simulink model "MOBATSim"  (R2020b)
settings: Solver=FixedStepAuto  StartTime=0.0  StopTime=Sim_t  FixedStep=0.01  MinStep=0.01  RelTol=1e-2
values from neighbouring files (symbols this model uses):
  Vehicles = evalin('base','Vehicles')    [I2V.m]    (also in VehicleSensors.m)
undefined symbols (not defined in the file or in its folder): Sim_Ts
libraries: simulink x50, robotalgslib x10, drivingvehiclecontroller x10, mpcadaslib x10, pid_lib x10
(part 6 of 7)

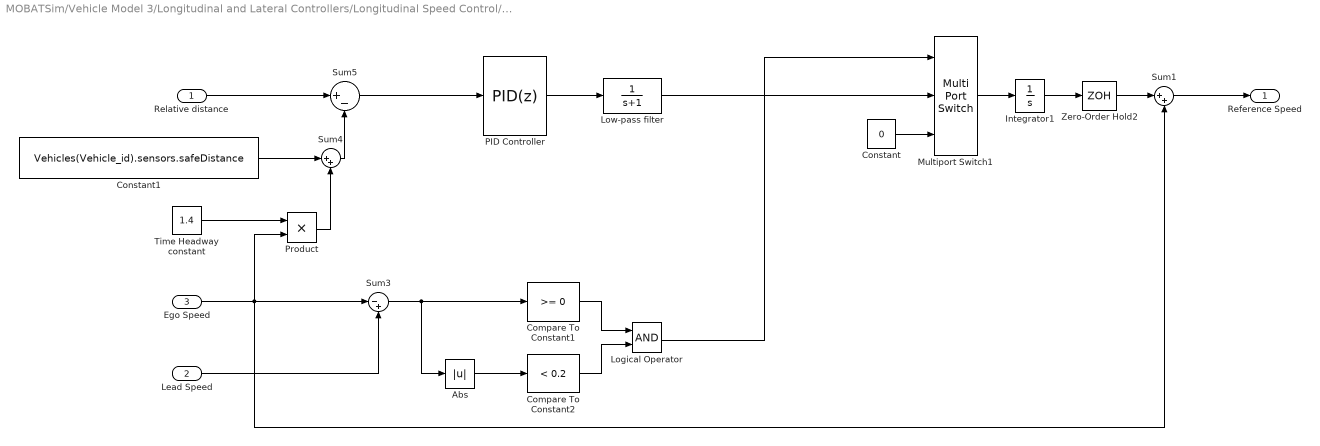
== system MOBATSim/Vehicle Model 3/Longitudinal and Lateral Controllers/Longitudinal Speed Control/Longitudinal Distance Control/PID-based ==
  Relative distance : Inport
  Lead Speed : Inport  Port=2
  Ego Speed : Inport  Port=3
  Abs : Abs
  Compare To Constant1 : simulink/Logic and Bit Operations/Compare To Constant  relop=>=  const=0  OutDataTypeStr=uint8
  Compare To Constant2 : simulink/Logic and Bit Operations/Compare To Constant  relop=<  const=0.2  OutDataTypeStr=uint8
  Constant : Constant  Value=0
  Constant1 : Constant  Value=Vehicles(Vehicle_id).sensors.safeDistance
  Integrator1 : Integrator  LimitOutput=on  UpperSaturationLimit=2  LowerSaturationLimit=-3
  Logical Operator : Logic  AllPortsSameDT=off  OutDataTypeStr=boolean
  Low-pass filter : TransferFcn  Denominator=[1 1]
  Multiport Switch1 : MultiPortSwitch  DataPortOrder=Zero-based contiguous  Inputs=2  zeroidx=on
  PID Controller : pid_lib/PID Controller  Controller=PID  Form=Parallel  TimeDomain=Discrete-time  UseExternalTs=off  SampleTime=0.1  IntegratorMethod=Trapezoidal  FilterMethod=Trapezoidal  ControllerParametersSource=internal  P=1.2  I=0.02  D=0.3  UseFilter=on  N=230  TunerSelectOption=Transfer Function Based (PID Tuner App)  InitialConditionSource=internal  InitialConditionForIntegrator=0  InitialConditionForFilter=0  DifferentiatorICPrevScaledInput=0  ExternalReset=none  TrackingMode=off  Kt=1  LimitOutput=on  SatLimitsSource=internal  UpperSaturationLimit=2  LowerSaturationLimit=-3  LinearizeAsGain=on  AntiWindupMode=back-calculation  Kb=1  POutMin=[]  POutMax=[]  IOutMin=[]  IOutMax=[]  DOutMin=[]  DOutMax=[]  NOutMin=[]  NOutMax=[]  SumOutMin=[]  SumOutMax=[]  SaturationOutMin=[]  SaturationOutMax=[]  PParamMin=[]  PParamMax=[]  IParamMin=[]  IParamMax=[]  DParamMin=[]  DParamMax=[]  NParamMin=[]  NParamMax=[]  KbParamMin=[]  KbParamMax=[]  KtParamMin=[]  KtParamMax=[]  KbOutMin=[]  KbOutMax=[]  KtOutMin=[]  KtOutMax=[]  IntegratorOutMin=[]  IntegratorOutMax=[]  FilterOutMin=[]  FilterOutMax=[]  SumI1OutMin=[]  SumI1OutMax=[]  SumI2OutMin=[]  SumI2OutMax=[]  SumI3OutMin=[]  SumI3OutMax=[]  SumI4OutMin=[]  SumI4OutMax=[]  SumDOutMin=[]  SumDOutMax=[]  DifferentiatorOutMin=[]  DifferentiatorOutMax=[]  FilterDiffOutCoefMin=[]  FilterDiffOutCoefMax=[]  ReciprocalOutMin=[]  ReciprocalOutMax=[]  SumDenOutMin=[]  SumDenOutMax=[]  SumNumOutMin=[]  SumNumOutMax=[]  DivideOutMin=[]  DivideOutMax=[]  UdiffTsProdOutMin=[]  UdiffTsProdOutMax=[]  NTsProdOutMin=[]  NTsProdOutMax=[]  UintegralTsProdOutMin=[]  UintegralTsProdOutMax=[]  UngainTsProdOutMin=[]  UngainTsProdOutMax=[]  IntegratorContinuousStateAttributes=''  IntegratorStateMustResolveToSignalObject=off  IntegratorRTWStateStorageClass=Auto  FilterContinuousStateAttributes=''  FilterStateMustResolveToSignalObject=off  FilterRTWStateStorageClass=Auto  ParallelPVariant=InternalParameters  IdealPVariant=Disabled  IVariant=InternalParameters  DVariant=InternalParameters  IntegratorVariant=Discrete  SatVariant=Enabled  AWVariant=BackCalculation  PCopyVariant=Disabled  TRVariant=Disabled  FdbkBlocksVariant=Feedback  IdealPFdbkVariant=Passthrough  SatFdbkVariant=Enabled  DerivativeFilterVariant=TrapezoidalFilter  NVariant=InternalParameters  NCopyVariant=InternalParameters  FilterICVariant=InternalICsFilter  IntegratorICVariant=InternalICs  ExternalResetVariant=Disabled  TRSumVariant=Passthrough  SumFdbkVariant=Enabled  SumVariant=Sum_PID  TsampFilterVariant=InternalTs  TsampNgainVariant=Passthrough  TsampIntegralVariant=Passthrough  ExternalSaturationOutDataTypeStr=Inherit: Same as second input
  Product : Product
  Sum1 : Sum  Inputs=|++
  Sum3 : Sum  Inputs=|-+
  Sum4 : Sum  Inputs=|++
  Sum5 : Sum  Inputs=|+-
  Time Headway constant : Constant  Value=1.4
  Zero-Order Hold2 : ZeroOrderHold  SampleTime=Sim_Ts
  Reference Speed : Outport  VectorParamsAs1DForOutWhenUnconnected=off
  wires:
  Low-pass filter/1 -> Multiport Switch1/2
  Lead Speed/1 -> Sum3/2
  PID Controller/1 -> Low-pass filter/1
  Time Headway constant/1 -> Product/1
  Constant1/1 -> Sum4/1
  Sum4/1 -> Sum5/2
  Abs/1 -> Compare To Constant2/1
  Logical Operator/1 -> Multiport Switch1/1
  Compare To Constant2/1 -> Logical Operator/2
  Sum5/1 -> PID Controller/1
  Constant/1 -> Multiport Switch1/3
  Product/1 -> Sum4/2
  Relative distance/1 -> Sum5/1
  Sum3/1 -> Abs/1, Compare To Constant1/1
  Compare To Constant1/1 -> Logical Operator/1
  Zero-Order Hold2/1 -> Sum1/1
  Ego Speed/1 -> Product/2, Sum1/2, Sum3/1
  Integrator1/1 -> Zero-Order Hold2/1
  Multiport Switch1/1 -> Integrator1/1
  Sum1/1 -> Reference Speed/1

== system MOBATSim/Vehicle Model 4/Longitudinal and Lateral Controllers/Lateral Motion Control/Pure Pursuit/Wheel Steering Angle Formulation ==
  note: $\delta(t)=tan^{-1} \left( \frac{2\ L\ sin(\alpha)}{l_{d}} \right)$
  alpha : Inport
  Atan : Trigonometry  Operator=atan
  Divide : Product  Inputs=*/
  Gain : Gain  Gain=2
  One over Look Ahead Distance : Constant  Value=6
  Product : Product
  Sine Wave : Sin  TimeSource=Use external signal  SampleTime=0
  Wheel Base : Constant  Value=3
  referenceYawAngle : Outport
  wires:
  Wheel Base/1 -> Gain/1
  Gain/1 -> Product/1
  alpha/1 -> Sine Wave/1
  Sine Wave/1 -> Product/2
  Product/1 -> Divide/1
  One over Look Ahead Distance/1 -> Divide/2
  Divide/1 -> Atan/1
  Atan/1 -> referenceYawAngle/1

== system MOBATSim/Vehicle Model 4/Longitudinal and Lateral Controllers/Longitudinal Speed Control/Longitudinal Distance Control/MPC-based ==
  note: Needs Model Predictive Control Toolbox™ to run
  Relative distance : Inport
  Lead Speed : Inport  Port=2
  Ego Speed : Inport  Port=3
  Adaptive Cruise Control System : mpcadaslib/Adaptive Cruise Control System  EgoModel=tf(1,[1,0])  InitialEgoVelocity=0  DefaultSpacing=Vehicles(Vehicle_id).sensors.safeDistance  MaxVelocity=Vehicles(Vehicle_id).dynamics.maxSpeed  MinAcceleration=-3  amin_ext=off  MaxAcceleration=2  amax_ext=off  Ts=0.4  PredictionHorizon=5  ControllerBehavior=0.620  suboptimal=off  maxiter=10  datatypeopt=double  optmode=off  trackmode=off
  Constant1 : Constant  Value=1.4
  Constant2 : Constant  Value=Vehicles(Vehicle_id).dynamics.maxSpeed
  Integrator1 : Integrator  LimitOutput=on  UpperSaturationLimit=2  LowerSaturationLimit=-3
  Sum : Sum  Inputs=|-+
  Sum4 : Sum  Inputs=|++
  Zero-Order Hold2 : ZeroOrderHold  SampleTime=Sim_Ts
  Reference Speed : Outport  VectorParamsAs1DForOutWhenUnconnected=off
  wires:
  Sum/1 -> Adaptive Cruise Control System/5
  Relative distance/1 -> Adaptive Cruise Control System/4
  Adaptive Cruise Control System/1 -> Integrator1/1
  Integrator1/1 -> Zero-Order Hold2/1
  Sum4/1 -> Reference Speed/1
  Constant1/1 -> Adaptive Cruise Control System/2
  Constant2/1 -> Adaptive Cruise Control System/1
  Lead Speed/1 -> Sum/2
  Ego Speed/1 -> Sum4/2, Adaptive Cruise Control System/3, Sum/1
  Zero-Order Hold2/1 -> Sum4/1

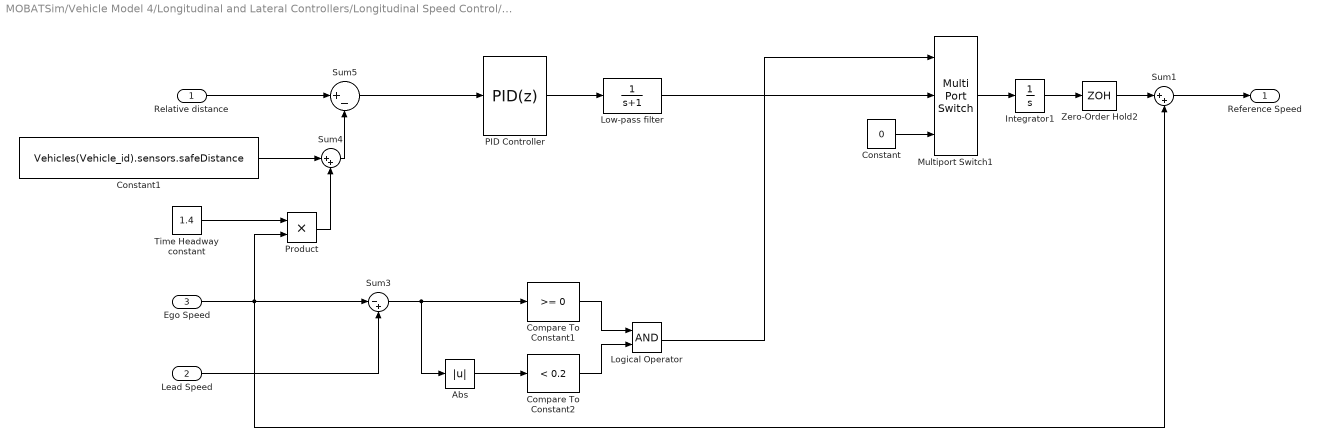
== system MOBATSim/Vehicle Model 4/Longitudinal and Lateral Controllers/Longitudinal Speed Control/Longitudinal Distance Control/PID-based ==
  Relative distance : Inport
  Lead Speed : Inport  Port=2
  Ego Speed : Inport  Port=3
  Abs : Abs
  Compare To Constant1 : simulink/Logic and Bit Operations/Compare To Constant  relop=>=  const=0  OutDataTypeStr=uint8
  Compare To Constant2 : simulink/Logic and Bit Operations/Compare To Constant  relop=<  const=0.2  OutDataTypeStr=uint8
  Constant : Constant  Value=0
  Constant1 : Constant  Value=Vehicles(Vehicle_id).sensors.safeDistance
  Integrator1 : Integrator  LimitOutput=on  UpperSaturationLimit=2  LowerSaturationLimit=-3
  Logical Operator : Logic  AllPortsSameDT=off  OutDataTypeStr=boolean
  Low-pass filter : TransferFcn  Denominator=[1 1]
  Multiport Switch1 : MultiPortSwitch  DataPortOrder=Zero-based contiguous  Inputs=2  zeroidx=on
  PID Controller : pid_lib/PID Controller  Controller=PID  Form=Parallel  TimeDomain=Discrete-time  UseExternalTs=off  SampleTime=0.1  IntegratorMethod=Trapezoidal  FilterMethod=Trapezoidal  ControllerParametersSource=internal  P=1.2  I=0.02  D=0.3  UseFilter=on  N=230  TunerSelectOption=Transfer Function Based (PID Tuner App)  InitialConditionSource=internal  InitialConditionForIntegrator=0  InitialConditionForFilter=0  DifferentiatorICPrevScaledInput=0  ExternalReset=none  TrackingMode=off  Kt=1  LimitOutput=on  SatLimitsSource=internal  UpperSaturationLimit=2  LowerSaturationLimit=-3  LinearizeAsGain=on  AntiWindupMode=back-calculation  Kb=1  POutMin=[]  POutMax=[]  IOutMin=[]  IOutMax=[]  DOutMin=[]  DOutMax=[]  NOutMin=[]  NOutMax=[]  SumOutMin=[]  SumOutMax=[]  SaturationOutMin=[]  SaturationOutMax=[]  PParamMin=[]  PParamMax=[]  IParamMin=[]  IParamMax=[]  DParamMin=[]  DParamMax=[]  NParamMin=[]  NParamMax=[]  KbParamMin=[]  KbParamMax=[]  KtParamMin=[]  KtParamMax=[]  KbOutMin=[]  KbOutMax=[]  KtOutMin=[]  KtOutMax=[]  IntegratorOutMin=[]  IntegratorOutMax=[]  FilterOutMin=[]  FilterOutMax=[]  SumI1OutMin=[]  SumI1OutMax=[]  SumI2OutMin=[]  SumI2OutMax=[]  SumI3OutMin=[]  SumI3OutMax=[]  SumI4OutMin=[]  SumI4OutMax=[]  SumDOutMin=[]  SumDOutMax=[]  DifferentiatorOutMin=[]  DifferentiatorOutMax=[]  FilterDiffOutCoefMin=[]  FilterDiffOutCoefMax=[]  ReciprocalOutMin=[]  ReciprocalOutMax=[]  SumDenOutMin=[]  SumDenOutMax=[]  SumNumOutMin=[]  SumNumOutMax=[]  DivideOutMin=[]  DivideOutMax=[]  UdiffTsProdOutMin=[]  UdiffTsProdOutMax=[]  NTsProdOutMin=[]  NTsProdOutMax=[]  UintegralTsProdOutMin=[]  UintegralTsProdOutMax=[]  UngainTsProdOutMin=[]  UngainTsProdOutMax=[]  IntegratorContinuousStateAttributes=''  IntegratorStateMustResolveToSignalObject=off  IntegratorRTWStateStorageClass=Auto  FilterContinuousStateAttributes=''  FilterStateMustResolveToSignalObject=off  FilterRTWStateStorageClass=Auto  ParallelPVariant=InternalParameters  IdealPVariant=Disabled  IVariant=InternalParameters  DVariant=InternalParameters  IntegratorVariant=Discrete  SatVariant=Enabled  AWVariant=BackCalculation  PCopyVariant=Disabled  TRVariant=Disabled  FdbkBlocksVariant=Feedback  IdealPFdbkVariant=Passthrough  SatFdbkVariant=Enabled  DerivativeFilterVariant=TrapezoidalFilter  NVariant=InternalParameters  NCopyVariant=InternalParameters  FilterICVariant=InternalICsFilter  IntegratorICVariant=InternalICs  ExternalResetVariant=Disabled  TRSumVariant=Passthrough  SumFdbkVariant=Enabled  SumVariant=Sum_PID  TsampFilterVariant=InternalTs  TsampNgainVariant=Passthrough  TsampIntegralVariant=Passthrough  ExternalSaturationOutDataTypeStr=Inherit: Same as second input
  Product : Product
  Sum1 : Sum  Inputs=|++
  Sum3 : Sum  Inputs=|-+
  Sum4 : Sum  Inputs=|++
  Sum5 : Sum  Inputs=|+-
  Time Headway constant : Constant  Value=1.4
  Zero-Order Hold2 : ZeroOrderHold  SampleTime=Sim_Ts
  Reference Speed : Outport  VectorParamsAs1DForOutWhenUnconnected=off
  wires:
  Low-pass filter/1 -> Multiport Switch1/2
  Lead Speed/1 -> Sum3/2
  PID Controller/1 -> Low-pass filter/1
  Time Headway constant/1 -> Product/1
  Constant1/1 -> Sum4/1
  Sum4/1 -> Sum5/2
  Abs/1 -> Compare To Constant2/1
  Logical Operator/1 -> Multiport Switch1/1
  Compare To Constant2/1 -> Logical Operator/2
  Sum5/1 -> PID Controller/1
  Constant/1 -> Multiport Switch1/3
  Product/1 -> Sum4/2
  Relative distance/1 -> Sum5/1
  Sum3/1 -> Abs/1, Compare To Constant1/1
  Compare To Constant1/1 -> Logical Operator/1
  Zero-Order Hold2/1 -> Sum1/1
  Ego Speed/1 -> Product/2, Sum1/2, Sum3/1
  Integrator1/1 -> Zero-Order Hold2/1
  Multiport Switch1/1 -> Integrator1/1
  Sum1/1 -> Reference Speed/1

== system MOBATSim/Vehicle Model 5/Longitudinal and Lateral Controllers/Lateral Motion Control/Pure Pursuit/Wheel Steering Angle Formulation ==
  note: $\delta(t)=tan^{-1} \left( \frac{2\ L\ sin(\alpha)}{l_{d}} \right)$
  alpha : Inport
  Atan : Trigonometry  Operator=atan
  Divide : Product  Inputs=*/
  Gain : Gain  Gain=2
  One over Look Ahead Distance : Constant  Value=6
  Product : Product
  Sine Wave : Sin  TimeSource=Use external signal  SampleTime=0
  Wheel Base : Constant  Value=3
  referenceYawAngle : Outport
  wires:
  Wheel Base/1 -> Gain/1
  Gain/1 -> Product/1
  alpha/1 -> Sine Wave/1
  Sine Wave/1 -> Product/2
  Product/1 -> Divide/1
  One over Look Ahead Distance/1 -> Divide/2
  Divide/1 -> Atan/1
  Atan/1 -> referenceYawAngle/1

== system MOBATSim/Vehicle Model 5/Longitudinal and Lateral Controllers/Longitudinal Speed Control/Longitudinal Distance Control/MPC-based ==
  note: Needs Model Predictive Control Toolbox™ to run
  Relative distance : Inport
  Lead Speed : Inport  Port=2
  Ego Speed : Inport  Port=3
  Adaptive Cruise Control System : mpcadaslib/Adaptive Cruise Control System  EgoModel=tf(1,[1,0])  InitialEgoVelocity=0  DefaultSpacing=Vehicles(Vehicle_id).sensors.safeDistance  MaxVelocity=Vehicles(Vehicle_id).dynamics.maxSpeed  MinAcceleration=-3  amin_ext=off  MaxAcceleration=2  amax_ext=off  Ts=0.4  PredictionHorizon=5  ControllerBehavior=0.620  suboptimal=off  maxiter=10  datatypeopt=double  optmode=off  trackmode=off
  Constant1 : Constant  Value=1.4
  Constant2 : Constant  Value=Vehicles(Vehicle_id).dynamics.maxSpeed
  Integrator1 : Integrator  LimitOutput=on  UpperSaturationLimit=2  LowerSaturationLimit=-3
  Sum : Sum  Inputs=|-+
  Sum4 : Sum  Inputs=|++
  Zero-Order Hold2 : ZeroOrderHold  SampleTime=Sim_Ts
  Reference Speed : Outport  VectorParamsAs1DForOutWhenUnconnected=off
  wires:
  Sum/1 -> Adaptive Cruise Control System/5
  Relative distance/1 -> Adaptive Cruise Control System/4
  Adaptive Cruise Control System/1 -> Integrator1/1
  Integrator1/1 -> Zero-Order Hold2/1
  Sum4/1 -> Reference Speed/1
  Constant1/1 -> Adaptive Cruise Control System/2
  Constant2/1 -> Adaptive Cruise Control System/1
  Lead Speed/1 -> Sum/2
  Ego Speed/1 -> Sum4/2, Adaptive Cruise Control System/3, Sum/1
  Zero-Order Hold2/1 -> Sum4/1

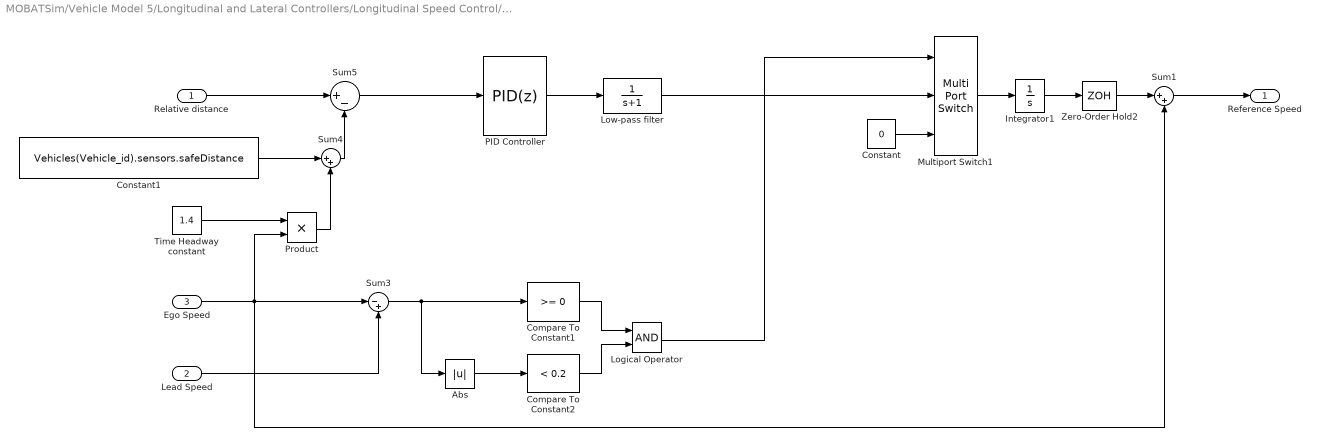
== system MOBATSim/Vehicle Model 5/Longitudinal and Lateral Controllers/Longitudinal Speed Control/Longitudinal Distance Control/PID-based ==
  Relative distance : Inport
  Lead Speed : Inport  Port=2
  Ego Speed : Inport  Port=3
  Abs : Abs
  Compare To Constant1 : simulink/Logic and Bit Operations/Compare To Constant  relop=>=  const=0  OutDataTypeStr=uint8
  Compare To Constant2 : simulink/Logic and Bit Operations/Compare To Constant  relop=<  const=0.2  OutDataTypeStr=uint8
  Constant : Constant  Value=0
  Constant1 : Constant  Value=Vehicles(Vehicle_id).sensors.safeDistance
  Integrator1 : Integrator  LimitOutput=on  UpperSaturationLimit=2  LowerSaturationLimit=-3
  Logical Operator : Logic  AllPortsSameDT=off  OutDataTypeStr=boolean
  Low-pass filter : TransferFcn  Denominator=[1 1]
  Multiport Switch1 : MultiPortSwitch  DataPortOrder=Zero-based contiguous  Inputs=2  zeroidx=on
  PID Controller : pid_lib/PID Controller  Controller=PID  Form=Parallel  TimeDomain=Discrete-time  UseExternalTs=off  SampleTime=0.1  IntegratorMethod=Trapezoidal  FilterMethod=Trapezoidal  ControllerParametersSource=internal  P=1.2  I=0.02  D=0.3  UseFilter=on  N=230  TunerSelectOption=Transfer Function Based (PID Tuner App)  InitialConditionSource=internal  InitialConditionForIntegrator=0  InitialConditionForFilter=0  DifferentiatorICPrevScaledInput=0  ExternalReset=none  TrackingMode=off  Kt=1  LimitOutput=on  SatLimitsSource=internal  UpperSaturationLimit=2  LowerSaturationLimit=-3  LinearizeAsGain=on  AntiWindupMode=back-calculation  Kb=1  POutMin=[]  POutMax=[]  IOutMin=[]  IOutMax=[]  DOutMin=[]  DOutMax=[]  NOutMin=[]  NOutMax=[]  SumOutMin=[]  SumOutMax=[]  SaturationOutMin=[]  SaturationOutMax=[]  PParamMin=[]  PParamMax=[]  IParamMin=[]  IParamMax=[]  DParamMin=[]  DParamMax=[]  NParamMin=[]  NParamMax=[]  KbParamMin=[]  KbParamMax=[]  KtParamMin=[]  KtParamMax=[]  KbOutMin=[]  KbOutMax=[]  KtOutMin=[]  KtOutMax=[]  IntegratorOutMin=[]  IntegratorOutMax=[]  FilterOutMin=[]  FilterOutMax=[]  SumI1OutMin=[]  SumI1OutMax=[]  SumI2OutMin=[]  SumI2OutMax=[]  SumI3OutMin=[]  SumI3OutMax=[]  SumI4OutMin=[]  SumI4OutMax=[]  SumDOutMin=[]  SumDOutMax=[]  DifferentiatorOutMin=[]  DifferentiatorOutMax=[]  FilterDiffOutCoefMin=[]  FilterDiffOutCoefMax=[]  ReciprocalOutMin=[]  ReciprocalOutMax=[]  SumDenOutMin=[]  SumDenOutMax=[]  SumNumOutMin=[]  SumNumOutMax=[]  DivideOutMin=[]  DivideOutMax=[]  UdiffTsProdOutMin=[]  UdiffTsProdOutMax=[]  NTsProdOutMin=[]  NTsProdOutMax=[]  UintegralTsProdOutMin=[]  UintegralTsProdOutMax=[]  UngainTsProdOutMin=[]  UngainTsProdOutMax=[]  IntegratorContinuousStateAttributes=''  IntegratorStateMustResolveToSignalObject=off  IntegratorRTWStateStorageClass=Auto  FilterContinuousStateAttributes=''  FilterStateMustResolveToSignalObject=off  FilterRTWStateStorageClass=Auto  ParallelPVariant=InternalParameters  IdealPVariant=Disabled  IVariant=InternalParameters  DVariant=InternalParameters  IntegratorVariant=Discrete  SatVariant=Enabled  AWVariant=BackCalculation  PCopyVariant=Disabled  TRVariant=Disabled  FdbkBlocksVariant=Feedback  IdealPFdbkVariant=Passthrough  SatFdbkVariant=Enabled  DerivativeFilterVariant=TrapezoidalFilter  NVariant=InternalParameters  NCopyVariant=InternalParameters  FilterICVariant=InternalICsFilter  IntegratorICVariant=InternalICs  ExternalResetVariant=Disabled  TRSumVariant=Passthrough  SumFdbkVariant=Enabled  SumVariant=Sum_PID  TsampFilterVariant=InternalTs  TsampNgainVariant=Passthrough  TsampIntegralVariant=Passthrough  ExternalSaturationOutDataTypeStr=Inherit: Same as second input
  Product : Product
  Sum1 : Sum  Inputs=|++
  Sum3 : Sum  Inputs=|-+
  Sum4 : Sum  Inputs=|++
  Sum5 : Sum  Inputs=|+-
  Time Headway constant : Constant  Value=1.4
  Zero-Order Hold2 : ZeroOrderHold  SampleTime=Sim_Ts
  Reference Speed : Outport  VectorParamsAs1DForOutWhenUnconnected=off
  wires:
  Low-pass filter/1 -> Multiport Switch1/2
  Lead Speed/1 -> Sum3/2
  PID Controller/1 -> Low-pass filter/1
  Time Headway constant/1 -> Product/1
  Constant1/1 -> Sum4/1
  Sum4/1 -> Sum5/2
  Abs/1 -> Compare To Constant2/1
  Logical Operator/1 -> Multiport Switch1/1
  Compare To Constant2/1 -> Logical Operator/2
  Sum5/1 -> PID Controller/1
  Constant/1 -> Multiport Switch1/3
  Product/1 -> Sum4/2
  Relative distance/1 -> Sum5/1
  Sum3/1 -> Abs/1, Compare To Constant1/1
  Compare To Constant1/1 -> Logical Operator/1
  Zero-Order Hold2/1 -> Sum1/1
  Ego Speed/1 -> Product/2, Sum1/2, Sum3/1
  Integrator1/1 -> Zero-Order Hold2/1
  Multiport Switch1/1 -> Integrator1/1
  Sum1/1 -> Reference Speed/1

== system MOBATSim/Vehicle Model 6/Longitudinal and Lateral Controllers/Lateral Motion Control/Pure Pursuit/Wheel Steering Angle Formulation ==
  note: $\delta(t)=tan^{-1} \left( \frac{2\ L\ sin(\alpha)}{l_{d}} \right)$
  alpha : Inport
  Atan : Trigonometry  Operator=atan
  Divide : Product  Inputs=*/
  Gain : Gain  Gain=2
  One over Look Ahead Distance : Constant  Value=6
  Product : Product
  Sine Wave : Sin  TimeSource=Use external signal  SampleTime=0
  Wheel Base : Constant  Value=3
  referenceYawAngle : Outport
  wires:
  Wheel Base/1 -> Gain/1
  Gain/1 -> Product/1
  alpha/1 -> Sine Wave/1
  Sine Wave/1 -> Product/2
  Product/1 -> Divide/1
  One over Look Ahead Distance/1 -> Divide/2
  Divide/1 -> Atan/1
  Atan/1 -> referenceYawAngle/1

== system MOBATSim/Vehicle Model 6/Longitudinal and Lateral Controllers/Longitudinal Speed Control/Longitudinal Distance Control/MPC-based ==
  note: Needs Model Predictive Control Toolbox™ to run
  Relative distance : Inport
  Lead Speed : Inport  Port=2
  Ego Speed : Inport  Port=3
  Adaptive Cruise Control System : mpcadaslib/Adaptive Cruise Control System  EgoModel=tf(1,[1,0])  InitialEgoVelocity=0  DefaultSpacing=Vehicles(Vehicle_id).sensors.safeDistance  MaxVelocity=Vehicles(Vehicle_id).dynamics.maxSpeed  MinAcceleration=-3  amin_ext=off  MaxAcceleration=2  amax_ext=off  Ts=0.4  PredictionHorizon=5  ControllerBehavior=0.620  suboptimal=off  maxiter=10  datatypeopt=double  optmode=off  trackmode=off
  Constant1 : Constant  Value=1.4
  Constant2 : Constant  Value=Vehicles(Vehicle_id).dynamics.maxSpeed
  Integrator1 : Integrator  LimitOutput=on  UpperSaturationLimit=2  LowerSaturationLimit=-3
  Sum : Sum  Inputs=|-+
  Sum4 : Sum  Inputs=|++
  Zero-Order Hold2 : ZeroOrderHold  SampleTime=Sim_Ts
  Reference Speed : Outport  VectorParamsAs1DForOutWhenUnconnected=off
  wires:
  Sum/1 -> Adaptive Cruise Control System/5
  Relative distance/1 -> Adaptive Cruise Control System/4
  Adaptive Cruise Control System/1 -> Integrator1/1
  Integrator1/1 -> Zero-Order Hold2/1
  Sum4/1 -> Reference Speed/1
  Constant1/1 -> Adaptive Cruise Control System/2
  Constant2/1 -> Adaptive Cruise Control System/1
  Lead Speed/1 -> Sum/2
  Ego Speed/1 -> Sum4/2, Adaptive Cruise Control System/3, Sum/1
  Zero-Order Hold2/1 -> Sum4/1

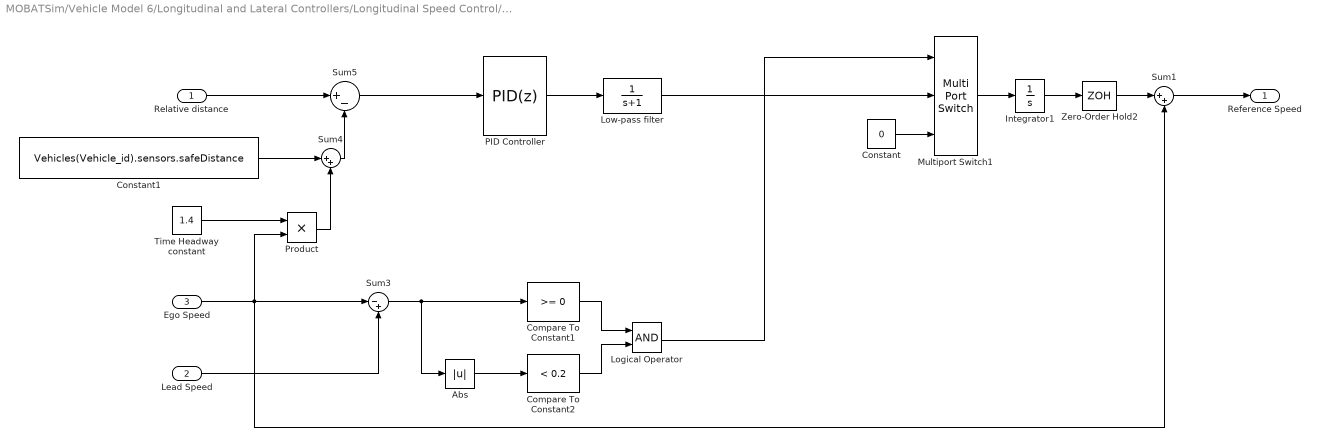
== system MOBATSim/Vehicle Model 6/Longitudinal and Lateral Controllers/Longitudinal Speed Control/Longitudinal Distance Control/PID-based ==
  Relative distance : Inport
  Lead Speed : Inport  Port=2
  Ego Speed : Inport  Port=3
  Abs : Abs
  Compare To Constant1 : simulink/Logic and Bit Operations/Compare To Constant  relop=>=  const=0  OutDataTypeStr=uint8
  Compare To Constant2 : simulink/Logic and Bit Operations/Compare To Constant  relop=<  const=0.2  OutDataTypeStr=uint8
  Constant : Constant  Value=0
  Constant1 : Constant  Value=Vehicles(Vehicle_id).sensors.safeDistance
  Integrator1 : Integrator  LimitOutput=on  UpperSaturationLimit=2  LowerSaturationLimit=-3
  Logical Operator : Logic  AllPortsSameDT=off  OutDataTypeStr=boolean
  Low-pass filter : TransferFcn  Denominator=[1 1]
  Multiport Switch1 : MultiPortSwitch  DataPortOrder=Zero-based contiguous  Inputs=2  zeroidx=on
  PID Controller : pid_lib/PID Controller  Controller=PID  Form=Parallel  TimeDomain=Discrete-time  UseExternalTs=off  SampleTime=0.1  IntegratorMethod=Trapezoidal  FilterMethod=Trapezoidal  ControllerParametersSource=internal  P=1.2  I=0.02  D=0.3  UseFilter=on  N=230  TunerSelectOption=Transfer Function Based (PID Tuner App)  InitialConditionSource=internal  InitialConditionForIntegrator=0  InitialConditionForFilter=0  DifferentiatorICPrevScaledInput=0  ExternalReset=none  TrackingMode=off  Kt=1  LimitOutput=on  SatLimitsSource=internal  UpperSaturationLimit=2  LowerSaturationLimit=-3  LinearizeAsGain=on  AntiWindupMode=back-calculation  Kb=1  POutMin=[]  POutMax=[]  IOutMin=[]  IOutMax=[]  DOutMin=[]  DOutMax=[]  NOutMin=[]  NOutMax=[]  SumOutMin=[]  SumOutMax=[]  SaturationOutMin=[]  SaturationOutMax=[]  PParamMin=[]  PParamMax=[]  IParamMin=[]  IParamMax=[]  DParamMin=[]  DParamMax=[]  NParamMin=[]  NParamMax=[]  KbParamMin=[]  KbParamMax=[]  KtParamMin=[]  KtParamMax=[]  KbOutMin=[]  KbOutMax=[]  KtOutMin=[]  KtOutMax=[]  IntegratorOutMin=[]  IntegratorOutMax=[]  FilterOutMin=[]  FilterOutMax=[]  SumI1OutMin=[]  SumI1OutMax=[]  SumI2OutMin=[]  SumI2OutMax=[]  SumI3OutMin=[]  SumI3OutMax=[]  SumI4OutMin=[]  SumI4OutMax=[]  SumDOutMin=[]  SumDOutMax=[]  DifferentiatorOutMin=[]  DifferentiatorOutMax=[]  FilterDiffOutCoefMin=[]  FilterDiffOutCoefMax=[]  ReciprocalOutMin=[]  ReciprocalOutMax=[]  SumDenOutMin=[]  SumDenOutMax=[]  SumNumOutMin=[]  SumNumOutMax=[]  DivideOutMin=[]  DivideOutMax=[]  UdiffTsProdOutMin=[]  UdiffTsProdOutMax=[]  NTsProdOutMin=[]  NTsProdOutMax=[]  UintegralTsProdOutMin=[]  UintegralTsProdOutMax=[]  UngainTsProdOutMin=[]  UngainTsProdOutMax=[]  IntegratorContinuousStateAttributes=''  IntegratorStateMustResolveToSignalObject=off  IntegratorRTWStateStorageClass=Auto  FilterContinuousStateAttributes=''  FilterStateMustResolveToSignalObject=off  FilterRTWStateStorageClass=Auto  ParallelPVariant=InternalParameters  IdealPVariant=Disabled  IVariant=InternalParameters  DVariant=InternalParameters  IntegratorVariant=Discrete  SatVariant=Enabled  AWVariant=BackCalculation  PCopyVariant=Disabled  TRVariant=Disabled  FdbkBlocksVariant=Feedback  IdealPFdbkVariant=Passthrough  SatFdbkVariant=Enabled  DerivativeFilterVariant=TrapezoidalFilter  NVariant=InternalParameters  NCopyVariant=InternalParameters  FilterICVariant=InternalICsFilter  IntegratorICVariant=InternalICs  ExternalResetVariant=Disabled  TRSumVariant=Passthrough  SumFdbkVariant=Enabled  SumVariant=Sum_PID  TsampFilterVariant=InternalTs  TsampNgainVariant=Passthrough  TsampIntegralVariant=Passthrough  ExternalSaturationOutDataTypeStr=Inherit: Same as second input
  Product : Product
  Sum1 : Sum  Inputs=|++
  Sum3 : Sum  Inputs=|-+
  Sum4 : Sum  Inputs=|++
  Sum5 : Sum  Inputs=|+-
  Time Headway constant : Constant  Value=1.4
  Zero-Order Hold2 : ZeroOrderHold  SampleTime=Sim_Ts
  Reference Speed : Outport  VectorParamsAs1DForOutWhenUnconnected=off
  wires:
  Low-pass filter/1 -> Multiport Switch1/2
  Lead Speed/1 -> Sum3/2
  PID Controller/1 -> Low-pass filter/1
  Time Headway constant/1 -> Product/1
  Constant1/1 -> Sum4/1
  Sum4/1 -> Sum5/2
  Abs/1 -> Compare To Constant2/1
  Logical Operator/1 -> Multiport Switch1/1
  Compare To Constant2/1 -> Logical Operator/2
  Sum5/1 -> PID Controller/1
  Constant/1 -> Multiport Switch1/3
  Product/1 -> Sum4/2
  Relative distance/1 -> Sum5/1
  Sum3/1 -> Abs/1, Compare To Constant1/1
  Compare To Constant1/1 -> Logical Operator/1
  Zero-Order Hold2/1 -> Sum1/1
  Ego Speed/1 -> Product/2, Sum1/2, Sum3/1
  Integrator1/1 -> Zero-Order Hold2/1
  Multiport Switch1/1 -> Integrator1/1
  Sum1/1 -> Reference Speed/1

== system MOBATSim/Vehicle Model 7/Longitudinal and Lateral Controllers/Lateral Motion Control/Pure Pursuit/Wheel Steering Angle Formulation ==
  note: $\delta(t)=tan^{-1} \left( \frac{2\ L\ sin(\alpha)}{l_{d}} \right)$
  alpha : Inport
  Atan : Trigonometry  Operator=atan
  Divide : Product  Inputs=*/
  Gain : Gain  Gain=2
  One over Look Ahead Distance : Constant  Value=6
  Product : Product
  Sine Wave : Sin  TimeSource=Use external signal  SampleTime=0
  Wheel Base : Constant  Value=3
  referenceYawAngle : Outport
  wires:
  Wheel Base/1 -> Gain/1
  Gain/1 -> Product/1
  alpha/1 -> Sine Wave/1
  Sine Wave/1 -> Product/2
  Product/1 -> Divide/1
  One over Look Ahead Distance/1 -> Divide/2
  Divide/1 -> Atan/1
  Atan/1 -> referenceYawAngle/1

== system MOBATSim/Vehicle Model 7/Longitudinal and Lateral Controllers/Longitudinal Speed Control/Longitudinal Distance Control/MPC-based ==
  note: Needs Model Predictive Control Toolbox™ to run
  Relative distance : Inport
  Lead Speed : Inport  Port=2
  Ego Speed : Inport  Port=3
  Adaptive Cruise Control System : mpcadaslib/Adaptive Cruise Control System  EgoModel=tf(1,[1,0])  InitialEgoVelocity=0  DefaultSpacing=Vehicles(Vehicle_id).sensors.safeDistance  MaxVelocity=Vehicles(Vehicle_id).dynamics.maxSpeed  MinAcceleration=-3  amin_ext=off  MaxAcceleration=2  amax_ext=off  Ts=0.4  PredictionHorizon=5  ControllerBehavior=0.620  suboptimal=off  maxiter=10  datatypeopt=double  optmode=off  trackmode=off
  Constant1 : Constant  Value=1.4
  Constant2 : Constant  Value=Vehicles(Vehicle_id).dynamics.maxSpeed
  Integrator1 : Integrator  LimitOutput=on  UpperSaturationLimit=2  LowerSaturationLimit=-3
  Sum : Sum  Inputs=|-+
  Sum4 : Sum  Inputs=|++
  Zero-Order Hold2 : ZeroOrderHold  SampleTime=Sim_Ts
  Reference Speed : Outport  VectorParamsAs1DForOutWhenUnconnected=off
  wires:
  Sum/1 -> Adaptive Cruise Control System/5
  Relative distance/1 -> Adaptive Cruise Control System/4
  Adaptive Cruise Control System/1 -> Integrator1/1
  Integrator1/1 -> Zero-Order Hold2/1
  Sum4/1 -> Reference Speed/1
  Constant1/1 -> Adaptive Cruise Control System/2
  Constant2/1 -> Adaptive Cruise Control System/1
  Lead Speed/1 -> Sum/2
  Ego Speed/1 -> Sum4/2, Adaptive Cruise Control System/3, Sum/1
  Zero-Order Hold2/1 -> Sum4/1

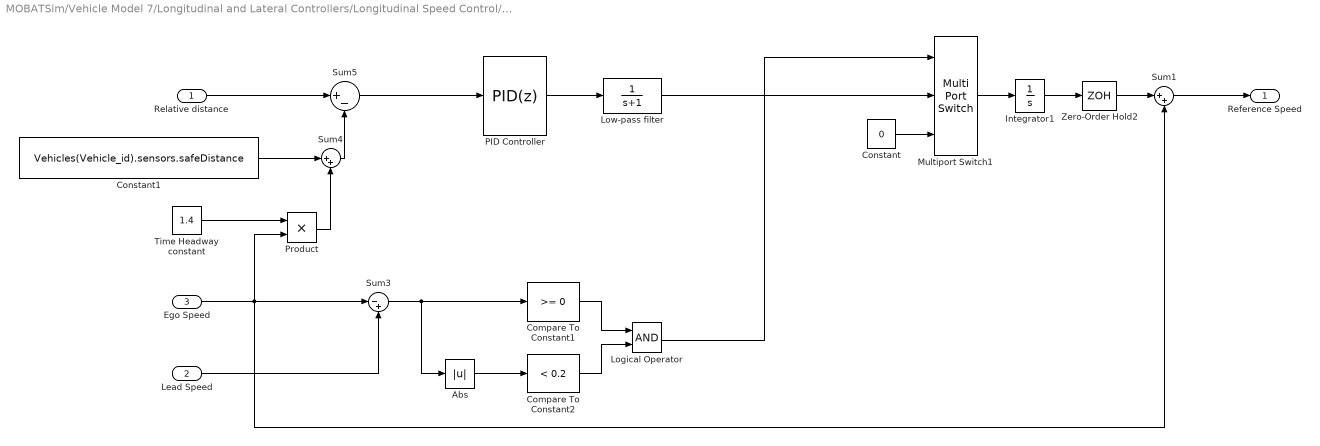
== system MOBATSim/Vehicle Model 7/Longitudinal and Lateral Controllers/Longitudinal Speed Control/Longitudinal Distance Control/PID-based ==
  Relative distance : Inport
  Lead Speed : Inport  Port=2
  Ego Speed : Inport  Port=3
  Abs : Abs
  Compare To Constant1 : simulink/Logic and Bit Operations/Compare To Constant  relop=>=  const=0  OutDataTypeStr=uint8
  Compare To Constant2 : simulink/Logic and Bit Operations/Compare To Constant  relop=<  const=0.2  OutDataTypeStr=uint8
  Constant : Constant  Value=0
  Constant1 : Constant  Value=Vehicles(Vehicle_id).sensors.safeDistance
  Integrator1 : Integrator  LimitOutput=on  UpperSaturationLimit=2  LowerSaturationLimit=-3
  Logical Operator : Logic  AllPortsSameDT=off  OutDataTypeStr=boolean
  Low-pass filter : TransferFcn  Denominator=[1 1]
  Multiport Switch1 : MultiPortSwitch  DataPortOrder=Zero-based contiguous  Inputs=2  zeroidx=on
  PID Controller : pid_lib/PID Controller  Controller=PID  Form=Parallel  TimeDomain=Discrete-time  UseExternalTs=off  SampleTime=0.1  IntegratorMethod=Trapezoidal  FilterMethod=Trapezoidal  ControllerParametersSource=internal  P=1.2  I=0.02  D=0.3  UseFilter=on  N=230  TunerSelectOption=Transfer Function Based (PID Tuner App)  InitialConditionSource=internal  InitialConditionForIntegrator=0  InitialConditionForFilter=0  DifferentiatorICPrevScaledInput=0  ExternalReset=none  TrackingMode=off  Kt=1  LimitOutput=on  SatLimitsSource=internal  UpperSaturationLimit=2  LowerSaturationLimit=-3  LinearizeAsGain=on  AntiWindupMode=back-calculation  Kb=1  POutMin=[]  POutMax=[]  IOutMin=[]  IOutMax=[]  DOutMin=[]  DOutMax=[]  NOutMin=[]  NOutMax=[]  SumOutMin=[]  SumOutMax=[]  SaturationOutMin=[]  SaturationOutMax=[]  PParamMin=[]  PParamMax=[]  IParamMin=[]  IParamMax=[]  DParamMin=[]  DParamMax=[]  NParamMin=[]  NParamMax=[]  KbParamMin=[]  KbParamMax=[]  KtParamMin=[]  KtParamMax=[]  KbOutMin=[]  KbOutMax=[]  KtOutMin=[]  KtOutMax=[]  IntegratorOutMin=[]  IntegratorOutMax=[]  FilterOutMin=[]  FilterOutMax=[]  SumI1OutMin=[]  SumI1OutMax=[]  SumI2OutMin=[]  SumI2OutMax=[]  SumI3OutMin=[]  SumI3OutMax=[]  SumI4OutMin=[]  SumI4OutMax=[]  SumDOutMin=[]  SumDOutMax=[]  DifferentiatorOutMin=[]  DifferentiatorOutMax=[]  FilterDiffOutCoefMin=[]  FilterDiffOutCoefMax=[]  ReciprocalOutMin=[]  ReciprocalOutMax=[]  SumDenOutMin=[]  SumDenOutMax=[]  SumNumOutMin=[]  SumNumOutMax=[]  DivideOutMin=[]  DivideOutMax=[]  UdiffTsProdOutMin=[]  UdiffTsProdOutMax=[]  NTsProdOutMin=[]  NTsProdOutMax=[]  UintegralTsProdOutMin=[]  UintegralTsProdOutMax=[]  UngainTsProdOutMin=[]  UngainTsProdOutMax=[]  IntegratorContinuousStateAttributes=''  IntegratorStateMustResolveToSignalObject=off  IntegratorRTWStateStorageClass=Auto  FilterContinuousStateAttributes=''  FilterStateMustResolveToSignalObject=off  FilterRTWStateStorageClass=Auto  ParallelPVariant=InternalParameters  IdealPVariant=Disabled  IVariant=InternalParameters  DVariant=InternalParameters  IntegratorVariant=Discrete  SatVariant=Enabled  AWVariant=BackCalculation  PCopyVariant=Disabled  TRVariant=Disabled  FdbkBlocksVariant=Feedback  IdealPFdbkVariant=Passthrough  SatFdbkVariant=Enabled  DerivativeFilterVariant=TrapezoidalFilter  NVariant=InternalParameters  NCopyVariant=InternalParameters  FilterICVariant=InternalICsFilter  IntegratorICVariant=InternalICs  ExternalResetVariant=Disabled  TRSumVariant=Passthrough  SumFdbkVariant=Enabled  SumVariant=Sum_PID  TsampFilterVariant=InternalTs  TsampNgainVariant=Passthrough  TsampIntegralVariant=Passthrough  ExternalSaturationOutDataTypeStr=Inherit: Same as second input
  Product : Product
  Sum1 : Sum  Inputs=|++
  Sum3 : Sum  Inputs=|-+
  Sum4 : Sum  Inputs=|++
  Sum5 : Sum  Inputs=|+-
  Time Headway constant : Constant  Value=1.4
  Zero-Order Hold2 : ZeroOrderHold  SampleTime=Sim_Ts
  Reference Speed : Outport  VectorParamsAs1DForOutWhenUnconnected=off
  wires:
  Low-pass filter/1 -> Multiport Switch1/2
  Lead Speed/1 -> Sum3/2
  PID Controller/1 -> Low-pass filter/1
  Time Headway constant/1 -> Product/1
  Constant1/1 -> Sum4/1
  Sum4/1 -> Sum5/2
  Abs/1 -> Compare To Constant2/1
  Logical Operator/1 -> Multiport Switch1/1
  Compare To Constant2/1 -> Logical Operator/2
  Sum5/1 -> PID Controller/1
  Constant/1 -> Multiport Switch1/3
  Product/1 -> Sum4/2
  Relative distance/1 -> Sum5/1
  Sum3/1 -> Abs/1, Compare To Constant1/1
  Compare To Constant1/1 -> Logical Operator/1
  Zero-Order Hold2/1 -> Sum1/1
  Ego Speed/1 -> Product/2, Sum1/2, Sum3/1
  Integrator1/1 -> Zero-Order Hold2/1
  Multiport Switch1/1 -> Integrator1/1
  Sum1/1 -> Reference Speed/1

== system MOBATSim/Vehicle Model 8/Longitudinal and Lateral Controllers/Lateral Motion Control/Pure Pursuit/Wheel Steering Angle Formulation ==
  note: $\delta(t)=tan^{-1} \left( \frac{2\ L\ sin(\alpha)}{l_{d}} \right)$
  alpha : Inport
  Atan : Trigonometry  Operator=atan
  Divide : Product  Inputs=*/
  Gain : Gain  Gain=2
  One over Look Ahead Distance : Constant  Value=6
  Product : Product
  Sine Wave : Sin  TimeSource=Use external signal  SampleTime=0
  Wheel Base : Constant  Value=3
  referenceYawAngle : Outport
  wires:
  Wheel Base/1 -> Gain/1
  Gain/1 -> Product/1
  alpha/1 -> Sine Wave/1
  Sine Wave/1 -> Product/2
  Product/1 -> Divide/1
  One over Look Ahead Distance/1 -> Divide/2
  Divide/1 -> Atan/1
  Atan/1 -> referenceYawAngle/1

== system MOBATSim/Vehicle Model 8/Longitudinal and Lateral Controllers/Longitudinal Speed Control/Longitudinal Distance Control/MPC-based ==
  note: Needs Model Predictive Control Toolbox™ to run
  Relative distance : Inport
  Lead Speed : Inport  Port=2
  Ego Speed : Inport  Port=3
  Adaptive Cruise Control System : mpcadaslib/Adaptive Cruise Control System  EgoModel=tf(1,[1,0])  InitialEgoVelocity=0  DefaultSpacing=Vehicles(Vehicle_id).sensors.safeDistance  MaxVelocity=Vehicles(Vehicle_id).dynamics.maxSpeed  MinAcceleration=-3  amin_ext=off  MaxAcceleration=2  amax_ext=off  Ts=0.4  PredictionHorizon=5  ControllerBehavior=0.620  suboptimal=off  maxiter=10  datatypeopt=double  optmode=off  trackmode=off
  Constant1 : Constant  Value=1.4
  Constant2 : Constant  Value=Vehicles(Vehicle_id).dynamics.maxSpeed
  Integrator1 : Integrator  LimitOutput=on  UpperSaturationLimit=2  LowerSaturationLimit=-3
  Sum : Sum  Inputs=|-+
  Sum4 : Sum  Inputs=|++
  Zero-Order Hold2 : ZeroOrderHold  SampleTime=Sim_Ts
  Reference Speed : Outport  VectorParamsAs1DForOutWhenUnconnected=off
  wires:
  Sum/1 -> Adaptive Cruise Control System/5
  Relative distance/1 -> Adaptive Cruise Control System/4
  Adaptive Cruise Control System/1 -> Integrator1/1
  Integrator1/1 -> Zero-Order Hold2/1
  Sum4/1 -> Reference Speed/1
  Constant1/1 -> Adaptive Cruise Control System/2
  Constant2/1 -> Adaptive Cruise Control System/1
  Lead Speed/1 -> Sum/2
  Ego Speed/1 -> Sum4/2, Adaptive Cruise Control System/3, Sum/1
  Zero-Order Hold2/1 -> Sum4/1

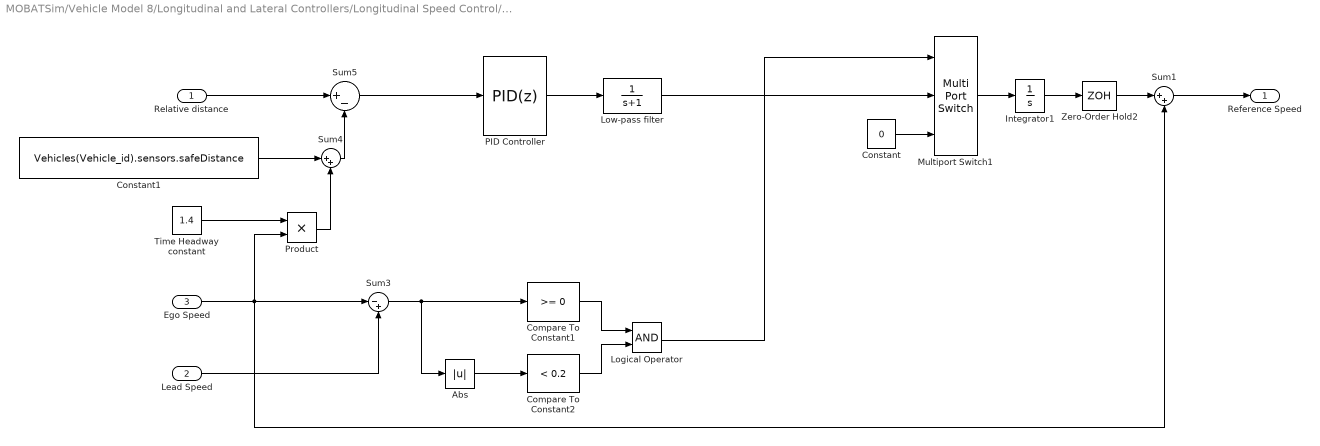
== system MOBATSim/Vehicle Model 8/Longitudinal and Lateral Controllers/Longitudinal Speed Control/Longitudinal Distance Control/PID-based ==
  Relative distance : Inport
  Lead Speed : Inport  Port=2
  Ego Speed : Inport  Port=3
  Abs : Abs
  Compare To Constant1 : simulink/Logic and Bit Operations/Compare To Constant  relop=>=  const=0  OutDataTypeStr=uint8
  Compare To Constant2 : simulink/Logic and Bit Operations/Compare To Constant  relop=<  const=0.2  OutDataTypeStr=uint8
  Constant : Constant  Value=0
  Constant1 : Constant  Value=Vehicles(Vehicle_id).sensors.safeDistance
  Integrator1 : Integrator  LimitOutput=on  UpperSaturationLimit=2  LowerSaturationLimit=-3
  Logical Operator : Logic  AllPortsSameDT=off  OutDataTypeStr=boolean
  Low-pass filter : TransferFcn  Denominator=[1 1]
  Multiport Switch1 : MultiPortSwitch  DataPortOrder=Zero-based contiguous  Inputs=2  zeroidx=on
  PID Controller : pid_lib/PID Controller  Controller=PID  Form=Parallel  TimeDomain=Discrete-time  UseExternalTs=off  SampleTime=0.1  IntegratorMethod=Trapezoidal  FilterMethod=Trapezoidal  ControllerParametersSource=internal  P=1.2  I=0.02  D=0.3  UseFilter=on  N=230  TunerSelectOption=Transfer Function Based (PID Tuner App)  InitialConditionSource=internal  InitialConditionForIntegrator=0  InitialConditionForFilter=0  DifferentiatorICPrevScaledInput=0  ExternalReset=none  TrackingMode=off  Kt=1  LimitOutput=on  SatLimitsSource=internal  UpperSaturationLimit=2  LowerSaturationLimit=-3  LinearizeAsGain=on  AntiWindupMode=back-calculation  Kb=1  POutMin=[]  POutMax=[]  IOutMin=[]  IOutMax=[]  DOutMin=[]  DOutMax=[]  NOutMin=[]  NOutMax=[]  SumOutMin=[]  SumOutMax=[]  SaturationOutMin=[]  SaturationOutMax=[]  PParamMin=[]  PParamMax=[]  IParamMin=[]  IParamMax=[]  DParamMin=[]  DParamMax=[]  NParamMin=[]  NParamMax=[]  KbParamMin=[]  KbParamMax=[]  KtParamMin=[]  KtParamMax=[]  KbOutMin=[]  KbOutMax=[]  KtOutMin=[]  KtOutMax=[]  IntegratorOutMin=[]  IntegratorOutMax=[]  FilterOutMin=[]  FilterOutMax=[]  SumI1OutMin=[]  SumI1OutMax=[]  SumI2OutMin=[]  SumI2OutMax=[]  SumI3OutMin=[]  SumI3OutMax=[]  SumI4OutMin=[]  SumI4OutMax=[]  SumDOutMin=[]  SumDOutMax=[]  DifferentiatorOutMin=[]  DifferentiatorOutMax=[]  FilterDiffOutCoefMin=[]  FilterDiffOutCoefMax=[]  ReciprocalOutMin=[]  ReciprocalOutMax=[]  SumDenOutMin=[]  SumDenOutMax=[]  SumNumOutMin=[]  SumNumOutMax=[]  DivideOutMin=[]  DivideOutMax=[]  UdiffTsProdOutMin=[]  UdiffTsProdOutMax=[]  NTsProdOutMin=[]  NTsProdOutMax=[]  UintegralTsProdOutMin=[]  UintegralTsProdOutMax=[]  UngainTsProdOutMin=[]  UngainTsProdOutMax=[]  IntegratorContinuousStateAttributes=''  IntegratorStateMustResolveToSignalObject=off  IntegratorRTWStateStorageClass=Auto  FilterContinuousStateAttributes=''  FilterStateMustResolveToSignalObject=off  FilterRTWStateStorageClass=Auto  ParallelPVariant=InternalParameters  IdealPVariant=Disabled  IVariant=InternalParameters  DVariant=InternalParameters  IntegratorVariant=Discrete  SatVariant=Enabled  AWVariant=BackCalculation  PCopyVariant=Disabled  TRVariant=Disabled  FdbkBlocksVariant=Feedback  IdealPFdbkVariant=Passthrough  SatFdbkVariant=Enabled  DerivativeFilterVariant=TrapezoidalFilter  NVariant=InternalParameters  NCopyVariant=InternalParameters  FilterICVariant=InternalICsFilter  IntegratorICVariant=InternalICs  ExternalResetVariant=Disabled  TRSumVariant=Passthrough  SumFdbkVariant=Enabled  SumVariant=Sum_PID  TsampFilterVariant=InternalTs  TsampNgainVariant=Passthrough  TsampIntegralVariant=Passthrough  ExternalSaturationOutDataTypeStr=Inherit: Same as second input
  Product : Product
  Sum1 : Sum  Inputs=|++
  Sum3 : Sum  Inputs=|-+
  Sum4 : Sum  Inputs=|++
  Sum5 : Sum  Inputs=|+-
  Time Headway constant : Constant  Value=1.4
  Zero-Order Hold2 : ZeroOrderHold  SampleTime=Sim_Ts
  Reference Speed : Outport  VectorParamsAs1DForOutWhenUnconnected=off
  wires:
  Low-pass filter/1 -> Multiport Switch1/2
  Lead Speed/1 -> Sum3/2
  PID Controller/1 -> Low-pass filter/1
  Time Headway constant/1 -> Product/1
  Constant1/1 -> Sum4/1
  Sum4/1 -> Sum5/2
  Abs/1 -> Compare To Constant2/1
  Logical Operator/1 -> Multiport Switch1/1
  Compare To Constant2/1 -> Logical Operator/2
  Sum5/1 -> PID Controller/1
  Constant/1 -> Multiport Switch1/3
  Product/1 -> Sum4/2
  Relative distance/1 -> Sum5/1
  Sum3/1 -> Abs/1, Compare To Constant1/1
  Compare To Constant1/1 -> Logical Operator/1
  Zero-Order Hold2/1 -> Sum1/1
  Ego Speed/1 -> Product/2, Sum1/2, Sum3/1
  Integrator1/1 -> Zero-Order Hold2/1
  Multiport Switch1/1 -> Integrator1/1
  Sum1/1 -> Reference Speed/1

== system MOBATSim/Vehicle Model 9/Longitudinal and Lateral Controllers/Lateral Motion Control/Pure Pursuit/Wheel Steering Angle Formulation ==
  note: $\delta(t)=tan^{-1} \left( \frac{2\ L\ sin(\alpha)}{l_{d}} \right)$
  alpha : Inport
  Atan : Trigonometry  Operator=atan
  Divide : Product  Inputs=*/
  Gain : Gain  Gain=2
  One over Look Ahead Distance : Constant  Value=6
  Product : Product
  Sine Wave : Sin  TimeSource=Use external signal  SampleTime=0
  Wheel Base : Constant  Value=3
  referenceYawAngle : Outport
  wires:
  Wheel Base/1 -> Gain/1
  Gain/1 -> Product/1
  alpha/1 -> Sine Wave/1
  Sine Wave/1 -> Product/2
  Product/1 -> Divide/1
  One over Look Ahead Distance/1 -> Divide/2
  Divide/1 -> Atan/1
  Atan/1 -> referenceYawAngle/1

== system MOBATSim/Vehicle Model 9/Longitudinal and Lateral Controllers/Longitudinal Speed Control/Longitudinal Distance Control/MPC-based ==
  note: Needs Model Predictive Control Toolbox™ to run
  Relative distance : Inport
  Lead Speed : Inport  Port=2
  Ego Speed : Inport  Port=3
  Adaptive Cruise Control System : mpcadaslib/Adaptive Cruise Control System  EgoModel=tf(1,[1,0])  InitialEgoVelocity=0  DefaultSpacing=Vehicles(Vehicle_id).sensors.safeDistance  MaxVelocity=Vehicles(Vehicle_id).dynamics.maxSpeed  MinAcceleration=-3  amin_ext=off  MaxAcceleration=2  amax_ext=off  Ts=0.4  PredictionHorizon=5  ControllerBehavior=0.620  suboptimal=off  maxiter=10  datatypeopt=double  optmode=off  trackmode=off
  Constant1 : Constant  Value=1.4
  Constant2 : Constant  Value=Vehicles(Vehicle_id).dynamics.maxSpeed
  Integrator1 : Integrator  LimitOutput=on  UpperSaturationLimit=2  LowerSaturationLimit=-3
  Sum : Sum  Inputs=|-+
  Sum4 : Sum  Inputs=|++
  Zero-Order Hold2 : ZeroOrderHold  SampleTime=Sim_Ts
  Reference Speed : Outport  VectorParamsAs1DForOutWhenUnconnected=off
  wires:
  Sum/1 -> Adaptive Cruise Control System/5
  Relative distance/1 -> Adaptive Cruise Control System/4
  Adaptive Cruise Control System/1 -> Integrator1/1
  Integrator1/1 -> Zero-Order Hold2/1
  Sum4/1 -> Reference Speed/1
  Constant1/1 -> Adaptive Cruise Control System/2
  Constant2/1 -> Adaptive Cruise Control System/1
  Lead Speed/1 -> Sum/2
  Ego Speed/1 -> Sum4/2, Adaptive Cruise Control System/3, Sum/1
  Zero-Order Hold2/1 -> Sum4/1

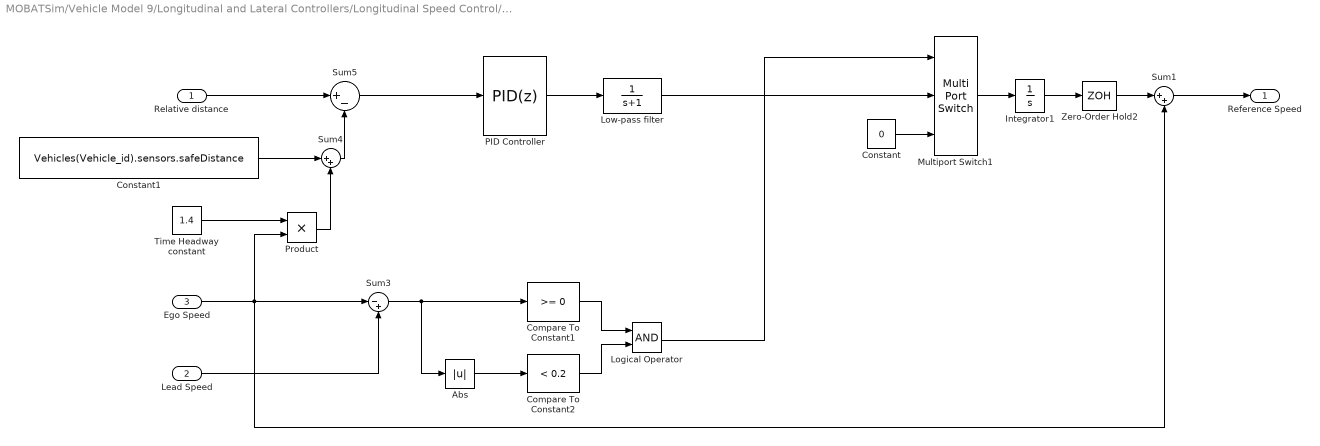
== system MOBATSim/Vehicle Model 9/Longitudinal and Lateral Controllers/Longitudinal Speed Control/Longitudinal Distance Control/PID-based ==
  Relative distance : Inport
  Lead Speed : Inport  Port=2
  Ego Speed : Inport  Port=3
  Abs : Abs
  Compare To Constant1 : simulink/Logic and Bit Operations/Compare To Constant  relop=>=  const=0  OutDataTypeStr=uint8
  Compare To Constant2 : simulink/Logic and Bit Operations/Compare To Constant  relop=<  const=0.2  OutDataTypeStr=uint8
  Constant : Constant  Value=0
  Constant1 : Constant  Value=Vehicles(Vehicle_id).sensors.safeDistance
  Integrator1 : Integrator  LimitOutput=on  UpperSaturationLimit=2  LowerSaturationLimit=-3
  Logical Operator : Logic  AllPortsSameDT=off  OutDataTypeStr=boolean
  Low-pass filter : TransferFcn  Denominator=[1 1]
  Multiport Switch1 : MultiPortSwitch  DataPortOrder=Zero-based contiguous  Inputs=2  zeroidx=on
  PID Controller : pid_lib/PID Controller  Controller=PID  Form=Parallel  TimeDomain=Discrete-time  UseExternalTs=off  SampleTime=0.1  IntegratorMethod=Trapezoidal  FilterMethod=Trapezoidal  ControllerParametersSource=internal  P=1.2  I=0.02  D=0.3  UseFilter=on  N=230  TunerSelectOption=Transfer Function Based (PID Tuner App)  InitialConditionSource=internal  InitialConditionForIntegrator=0  InitialConditionForFilter=0  DifferentiatorICPrevScaledInput=0  ExternalReset=none  TrackingMode=off  Kt=1  LimitOutput=on  SatLimitsSource=internal  UpperSaturationLimit=2  LowerSaturationLimit=-3  LinearizeAsGain=on  AntiWindupMode=back-calculation  Kb=1  POutMin=[]  POutMax=[]  IOutMin=[]  IOutMax=[]  DOutMin=[]  DOutMax=[]  NOutMin=[]  NOutMax=[]  SumOutMin=[]  SumOutMax=[]  SaturationOutMin=[]  SaturationOutMax=[]  PParamMin=[]  PParamMax=[]  IParamMin=[]  IParamMax=[]  DParamMin=[]  DParamMax=[]  NParamMin=[]  NParamMax=[]  KbParamMin=[]  KbParamMax=[]  KtParamMin=[]  KtParamMax=[]  KbOutMin=[]  KbOutMax=[]  KtOutMin=[]  KtOutMax=[]  IntegratorOutMin=[]  IntegratorOutMax=[]  FilterOutMin=[]  FilterOutMax=[]  SumI1OutMin=[]  SumI1OutMax=[]  SumI2OutMin=[]  SumI2OutMax=[]  SumI3OutMin=[]  SumI3OutMax=[]  SumI4OutMin=[]  SumI4OutMax=[]  SumDOutMin=[]  SumDOutMax=[]  DifferentiatorOutMin=[]  DifferentiatorOutMax=[]  FilterDiffOutCoefMin=[]  FilterDiffOutCoefMax=[]  ReciprocalOutMin=[]  ReciprocalOutMax=[]  SumDenOutMin=[]  SumDenOutMax=[]  SumNumOutMin=[]  SumNumOutMax=[]  DivideOutMin=[]  DivideOutMax=[]  UdiffTsProdOutMin=[]  UdiffTsProdOutMax=[]  NTsProdOutMin=[]  NTsProdOutMax=[]  UintegralTsProdOutMin=[]  UintegralTsProdOutMax=[]  UngainTsProdOutMin=[]  UngainTsProdOutMax=[]  IntegratorContinuousStateAttributes=''  IntegratorStateMustResolveToSignalObject=off  IntegratorRTWStateStorageClass=Auto  FilterContinuousStateAttributes=''  FilterStateMustResolveToSignalObject=off  FilterRTWStateStorageClass=Auto  ParallelPVariant=InternalParameters  IdealPVariant=Disabled  IVariant=InternalParameters  DVariant=InternalParameters  IntegratorVariant=Discrete  SatVariant=Enabled  AWVariant=BackCalculation  PCopyVariant=Disabled  TRVariant=Disabled  FdbkBlocksVariant=Feedback  IdealPFdbkVariant=Passthrough  SatFdbkVariant=Enabled  DerivativeFilterVariant=TrapezoidalFilter  NVariant=InternalParameters  NCopyVariant=InternalParameters  FilterICVariant=InternalICsFilter  IntegratorICVariant=InternalICs  ExternalResetVariant=Disabled  TRSumVariant=Passthrough  SumFdbkVariant=Enabled  SumVariant=Sum_PID  TsampFilterVariant=InternalTs  TsampNgainVariant=Passthrough  TsampIntegralVariant=Passthrough  ExternalSaturationOutDataTypeStr=Inherit: Same as second input
  Product : Product
  Sum1 : Sum  Inputs=|++
  Sum3 : Sum  Inputs=|-+
  Sum4 : Sum  Inputs=|++
  Sum5 : Sum  Inputs=|+-
  Time Headway constant : Constant  Value=1.4
  Zero-Order Hold2 : ZeroOrderHold  SampleTime=Sim_Ts
  Reference Speed : Outport  VectorParamsAs1DForOutWhenUnconnected=off
  wires:
  Low-pass filter/1 -> Multiport Switch1/2
  Lead Speed/1 -> Sum3/2
  PID Controller/1 -> Low-pass filter/1
  Time Headway constant/1 -> Product/1
  Constant1/1 -> Sum4/1
  Sum4/1 -> Sum5/2
  Abs/1 -> Compare To Constant2/1
  Logical Operator/1 -> Multiport Switch1/1
  Compare To Constant2/1 -> Logical Operator/2
  Sum5/1 -> PID Controller/1
  Constant/1 -> Multiport Switch1/3
  Product/1 -> Sum4/2
  Relative distance/1 -> Sum5/1
  Sum3/1 -> Abs/1, Compare To Constant1/1
  Compare To Constant1/1 -> Logical Operator/1
  Zero-Order Hold2/1 -> Sum1/1
  Ego Speed/1 -> Product/2, Sum1/2, Sum3/1
  Integrator1/1 -> Zero-Order Hold2/1
  Multiport Switch1/1 -> Integrator1/1
  Sum1/1 -> Reference Speed/1

== matlab function MOBATSim/Vehicle Model 3/Longitudinal and Lateral Controllers/Longitudinal Speed Control/Reference Acceleration Generation/Simple Gear Logic ==
  data: speed input; maxAcc output
function maxAcc = fcn(speed)
% Simple gear logic

    if speed < 3
        maxAcc = 6;
    
    elseif speed >= 3 && speed < 6
        maxAcc = 5;
        
    elseif speed >= 6 && speed < 9
        maxAcc = 3.8;
        
    elseif speed >= 9 && speed < 12
        maxAcc = 3;
        
    elseif speed >= 12 && speed < 14
        maxAcc = 2.2;
    else
        % if speed is greater than 14
        maxAcc = 1.4;  
    end

end

== matlab function MOBATSim/Vehicle Model 4/Longitudinal and Lateral Controllers/Longitudinal Speed Control/Reference Acceleration Generation/Simple Gear Logic ==
  data: speed input; maxAcc output
function maxAcc = fcn(speed)
% Simple gear logic

    if speed < 3
        maxAcc = 6;
    
    elseif speed >= 3 && speed < 6
        maxAcc = 5;
        
    elseif speed >= 6 && speed < 9
        maxAcc = 3.8;
        
    elseif speed >= 9 && speed < 12
        maxAcc = 3;
        
    elseif speed >= 12 && speed < 14
        maxAcc = 2.2;
    else
        % if speed is greater than 14
        maxAcc = 1.4;  
    end

end

== matlab function MOBATSim/Vehicle Model 5/Longitudinal and Lateral Controllers/Longitudinal Speed Control/Reference Acceleration Generation/Simple Gear Logic ==
  data: speed input; maxAcc output
function maxAcc = fcn(speed)
% Simple gear logic

    if speed < 3
        maxAcc = 6;
    
    elseif speed >= 3 && speed < 6
        maxAcc = 5;
        
    elseif speed >= 6 && speed < 9
        maxAcc = 3.8;
        
    elseif speed >= 9 && speed < 12
        maxAcc = 3;
        
    elseif speed >= 12 && speed < 14
        maxAcc = 2.2;
    else
        % if speed is greater than 14
        maxAcc = 1.4;  
    end

end

== matlab function MOBATSim/Vehicle Model 6/Longitudinal and Lateral Controllers/Longitudinal Speed Control/Reference Acceleration Generation/Simple Gear Logic ==
  data: speed input; maxAcc output
function maxAcc = fcn(speed)
% Simple gear logic

    if speed < 3
        maxAcc = 6;
    
    elseif speed >= 3 && speed < 6
        maxAcc = 5;
        
    elseif speed >= 6 && speed < 9
        maxAcc = 3.8;
        
    elseif speed >= 9 && speed < 12
        maxAcc = 3;
        
    elseif speed >= 12 && speed < 14
        maxAcc = 2.2;
    else
        % if speed is greater than 14
        maxAcc = 1.4;  
    end

end

== matlab function MOBATSim/Vehicle Model 7/Longitudinal and Lateral Controllers/Longitudinal Speed Control/Reference Acceleration Generation/Simple Gear Logic ==
  data: speed input; maxAcc output
function maxAcc = fcn(speed)
% Simple gear logic

    if speed < 3
        maxAcc = 6;
    
    elseif speed >= 3 && speed < 6
        maxAcc = 5;
        
    elseif speed >= 6 && speed < 9
        maxAcc = 3.8;
        
    elseif speed >= 9 && speed < 12
        maxAcc = 3;
        
    elseif speed >= 12 && speed < 14
        maxAcc = 2.2;
    else
        % if speed is greater than 14
        maxAcc = 1.4;  
    end

end
